simulink model "writeWord"  (Simulink 7.6)
settings: Solver=FixedStepDiscrete  StartTime=0.0  StopTime=10.0  FixedStep=0.001  RelTol=1e-3
libraries: simulink x17, dsPICdrivers x6
settings Model: Creator=ij8977  LastModifiedBy=ij8977
settings OptimizationCC: OptimizeModelRefInitCode=on  LifeSpan=1
settings RTWCC: SystemTargetFile=pic32.tlc  TemplateMakefile=pic32_gcc.tmf  PostCodeGenCommand=dsPIC_Compile()  Description=Embedded Target for Microchip dsPIC (real-time)  ProcessScript=pic32_make_rtw_hook
settings CodeAppCC: IgnoreCustomStorageClasses=off
settings STFCustomTargetCC: IncludeMdlTerminateFcn=off  CombineOutputUpdateFcns=on  SuppressErrorStatus=on  ERTCustomFileBanners=on  SupportContinuousTime=off  SupportNonInlinedSFcns=off  SystemTargetFile=pic32.tlc
settings ERTTargetCC: MultiwordLength=2048  ParMdlRefBuildCompliant=off  CompOptLevelCompliant=off  IncludeMdlTerminateFcn=off  SuppressErrorStatus=on  ERTFirstTimeCompliant=off  ModelStepFunctionPrototypeControlCompliant=off  CPPClassGenCompliant=off  InlinedParameterPlacement=NonHierarchical  ERTSrcFileBannerTemplate=dsPIC_code_template.cgt  ERTHdrFileBannerTemplate=dsPIC_code_template.cgt  ERTDataSrcFileTemplate=dsPIC_code_template.cgt  ERTDataHdrFileTemplate=dsPIC_code_template.cgt  ERTCustomFileTemplate=dsPIC_main.tlc  ConvertIfToSwitch=off
settings CustomProperty: DataType=string  Value=C:\PROGRA~1\MATLAB\R2010b\bin\win32\gmake

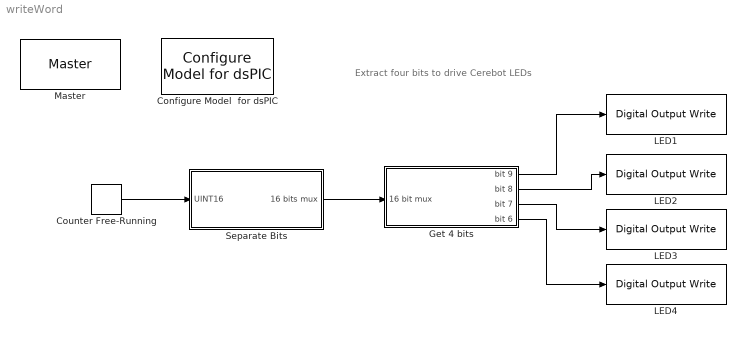
== system writeWord ==
  note: Extract four bits to drive Cerebot LEDs
  Configure Model  for dsPIC : dsPICdrivers/Simulink Configuration/Configure Model  for dsPIC
  Counter Free-Running : simulink/Sources/Counter Free-Running  SystemSampleTime=-1  NumBits=16  tsamp=-1
  Get 4 bits : Subsystem
  LED1 : dsPICdrivers/Digital I//O/Digital Output Write  Tag=dsPIC_Digital_Output  Priority=5  PORT=B  Pin=[10]  Simultaneous=off  OrderingInOutPopup=None
  LED2 : dsPICdrivers/Digital I//O/Digital Output Write  Tag=dsPIC_Digital_Output  Priority=5  PORT=B  Pin=[11]  Simultaneous=off  OrderingInOutPopup=None
  LED3 : dsPICdrivers/Digital I//O/Digital Output Write  Tag=dsPIC_Digital_Output  Priority=5  PORT=B  Pin=[12]  Simultaneous=off  OrderingInOutPopup=None
  LED4 : dsPICdrivers/Digital I//O/Digital Output Write  Tag=dsPIC_Digital_Output  Priority=5  PORT=B  Pin=[13]  Simultaneous=off  OrderingInOutPopup=None
  Master : dsPICdrivers/Master  Tag=dsPIC_MASTER  Priority=1  TimeStepType=Timer1  picType=32MX460F512L  fcy=80000000  Quartz_33f=8e6  PLLActive_33f=on  fcyDesired_33f=80e6  tmr1="[8  9999  0]"  tmr1Info="Time Step : 0.001  ;   Error : 0%  PR1=9999"  tmr2345="[0  0  0  0]"  tmr2345cfg=[-1 -1 -1 -1]  IOautoConf=on  typePort="[ 0   0   0   0   0   0   0   0   0   0   0   0   0   0   0   0   0   0   0   0   0   0   0   0   0   0  10  10  10  10   0   0   0   0   0   0   0   0   0   0   0   0   0   0   0   0   0   0   0   0   0   0   0   0   0   0   0   0   0   0   0   0   0   0   0   0   0   0   0   0   0   0   0   0   0   0   0   0   0   0   0   0   0   0   0   0   0   0   0   0   0   0   0   0   0   0   0   0   0   0   0   0   0   0   0   0   0   0   0   0   0   0 ]"  TRIS="[ 65535  50175  65535  65535  65535  65535  65535 ]"  ADPCFG=15360  MasterBusyPort=None  MasterOverloadPort=None  FOSC=Quartz (XT - HS)  ClockSwitchMonitor=Both disabled  TempProtection_33f=TEMP_ON  FPBOR=<empty>  PWRT=disable  MCLR=<empty>  ICD=ICS_NONE  JTAGEN=JTAGEN_OFF  PowerSave=off  OverrideFcy=off  NewFcy=1e6  PR2345="[65535  65535  65535  65535]"
  Separate Bits : Subsystem
  wires:
  Counter Free-Running/1 -> Separate Bits/1(UINT16)
  Get 4 bits/1(bit 9) -> LED1/1
  Get 4 bits/2(bit 8) -> LED2/1
  Get 4 bits/3(bit 7) -> LED3/1
  Get 4 bits/4(bit 6) -> LED4/1
  Separate Bits/1(16 bits mux) -> Get 4 bits/1(16 bit mux)

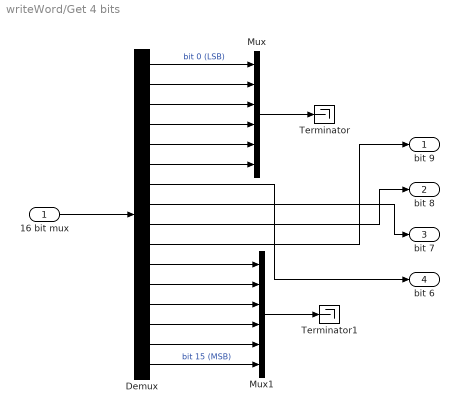
== system writeWord/Get 4 bits ==
  16 bit mux : Inport
  Demux : Demux  Outputs=16
  Mux : Mux  Inputs=6
  Mux1 : Mux  Inputs=6
  Terminator : Terminator
  Terminator1 : Terminator
  bit 9 : Outport
  bit 8 : Outport  Port=2
  bit 7 : Outport  Port=3
  bit 6 : Outport  Port=4
  wires:
  Mux/1 -> Terminator/1
  Demux/1 -> Mux/1  "bit 0 (LSB)"
  Demux/2 -> Mux/2
  Demux/3 -> Mux/3
  Demux/4 -> Mux/4
  Demux/5 -> Mux/5
  Demux/6 -> Mux/6
  Mux1/1 -> Terminator1/1
  Demux/11 -> Mux1/1
  Demux/12 -> Mux1/2
  Demux/13 -> Mux1/3
  Demux/14 -> Mux1/4
  Demux/15 -> Mux1/5
  Demux/16 -> Mux1/6  "bit 15 (MSB)"
  Demux/7 -> bit 6/1
  Demux/8 -> bit 7/1
  Demux/9 -> bit 8/1
  Demux/10 -> bit 9/1
  16 bit mux/1 -> Demux/1

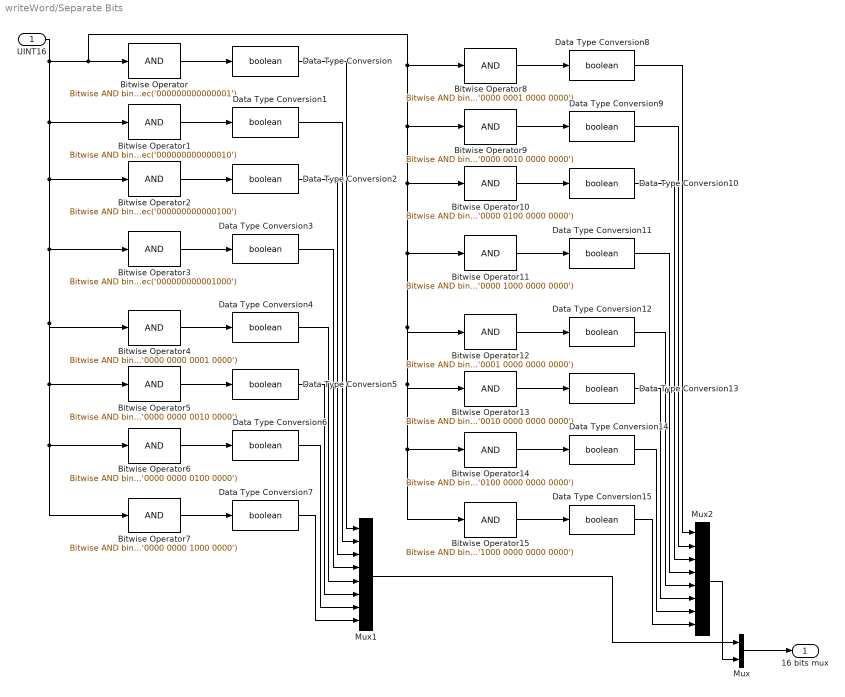
== system writeWord/Separate Bits ==
  UINT16 : Inport
  Bitwise Operator : simulink/Logic and Bit Operations/Bitwise Operator  logicop=AND  UseBitMask=on  BitMask=bin2dec('000000000000001')  BitMaskRealWorld=Stored Integer
  Bitwise Operator1 : simulink/Logic and Bit Operations/Bitwise Operator  logicop=AND  UseBitMask=on  BitMask=bin2dec('000000000000010')  BitMaskRealWorld=Stored Integer
  Bitwise Operator10 : simulink/Logic and Bit Operations/Bitwise Operator  logicop=AND  UseBitMask=on  BitMask=bin2dec('0000 0100 0000 0000')  BitMaskRealWorld=Stored Integer
  Bitwise Operator11 : simulink/Logic and Bit Operations/Bitwise Operator  logicop=AND  UseBitMask=on  BitMask=bin2dec('0000 1000 0000 0000')  BitMaskRealWorld=Stored Integer
  Bitwise Operator12 : simulink/Logic and Bit Operations/Bitwise Operator  logicop=AND  UseBitMask=on  BitMask=bin2dec('0001 0000 0000 0000')  BitMaskRealWorld=Stored Integer
  Bitwise Operator13 : simulink/Logic and Bit Operations/Bitwise Operator  logicop=AND  UseBitMask=on  BitMask=bin2dec('0010 0000 0000 0000')  BitMaskRealWorld=Stored Integer
  Bitwise Operator14 : simulink/Logic and Bit Operations/Bitwise Operator  logicop=AND  UseBitMask=on  BitMask=bin2dec('0100 0000 0000 0000')  BitMaskRealWorld=Stored Integer
  Bitwise Operator15 : simulink/Logic and Bit Operations/Bitwise Operator  logicop=AND  UseBitMask=on  BitMask=bin2dec('1000 0000 0000 0000')  BitMaskRealWorld=Stored Integer
  Bitwise Operator2 : simulink/Logic and Bit Operations/Bitwise Operator  logicop=AND  UseBitMask=on  BitMask=bin2dec('000000000000100')  BitMaskRealWorld=Stored Integer
  Bitwise Operator3 : simulink/Logic and Bit Operations/Bitwise Operator  logicop=AND  UseBitMask=on  BitMask=bin2dec('000000000001000')  BitMaskRealWorld=Stored Integer
  Bitwise Operator4 : simulink/Logic and Bit Operations/Bitwise Operator  logicop=AND  UseBitMask=on  BitMask=bin2dec('0000 0000 0001 0000')  BitMaskRealWorld=Stored Integer
  Bitwise Operator5 : simulink/Logic and Bit Operations/Bitwise Operator  logicop=AND  UseBitMask=on  BitMask=bin2dec('0000 0000 0010 0000')  BitMaskRealWorld=Stored Integer
  Bitwise Operator6 : simulink/Logic and Bit Operations/Bitwise Operator  logicop=AND  UseBitMask=on  BitMask=bin2dec('0000 0000 0100 0000')  BitMaskRealWorld=Stored Integer
  Bitwise Operator7 : simulink/Logic and Bit Operations/Bitwise Operator  logicop=AND  UseBitMask=on  BitMask=bin2dec('0000 0000 1000 0000')  BitMaskRealWorld=Stored Integer
  Bitwise Operator8 : simulink/Logic and Bit Operations/Bitwise Operator  logicop=AND  UseBitMask=on  BitMask=bin2dec('0000 0001 0000 0000')  BitMaskRealWorld=Stored Integer
  Bitwise Operator9 : simulink/Logic and Bit Operations/Bitwise Operator  logicop=AND  UseBitMask=on  BitMask=bin2dec('0000 0010 0000 0000')  BitMaskRealWorld=Stored Integer
  Data Type Conversion{,1..15} (16 alike) : DataTypeConversion  OutDataTypeStr=boolean
  Mux : Mux  Inputs=2
  Mux1 : Mux  Inputs=8
  Mux2 : Mux  Inputs=8
  16 bits mux : Outport
  wires:
  UINT16/1 -> Bitwise Operator1/1, Bitwise Operator7/1, Bitwise Operator6/1, Bitwise Operator5/1, Bitwise Operator4/1, Bitwise Operator3/1, Bitwise Operator2/1, Bitwise Operator/1, Bitwise Operator15/1, Bitwise Operator14/1, Bitwise Operator13/1, Bitwise Operator12/1, Bitwise Operator11/1, Bitwise Operator10/1, Bitwise Operator9/1, Bitwise Operator8/1
  Bitwise Operator/1 -> Data Type Conversion/1
  Data Type Conversion/1 -> Mux1/1
  Data Type Conversion1/1 -> Mux1/2
  Data Type Conversion2/1 -> Mux1/3
  Data Type Conversion3/1 -> Mux1/4
  Data Type Conversion4/1 -> Mux1/5
  Data Type Conversion5/1 -> Mux1/6
  Data Type Conversion6/1 -> Mux1/7
  Data Type Conversion7/1 -> Mux1/8
  Mux1/1 -> Mux/1
  Mux/1 -> 16 bits mux/1
  Bitwise Operator1/1 -> Data Type Conversion1/1
  Bitwise Operator2/1 -> Data Type Conversion2/1
  Bitwise Operator3/1 -> Data Type Conversion3/1
  Bitwise Operator4/1 -> Data Type Conversion4/1
  Bitwise Operator5/1 -> Data Type Conversion5/1
  Bitwise Operator6/1 -> Data Type Conversion6/1
  Bitwise Operator7/1 -> Data Type Conversion7/1
  Bitwise Operator8/1 -> Data Type Conversion8/1
  Data Type Conversion8/1 -> Mux2/1
  Data Type Conversion9/1 -> Mux2/2
  Data Type Conversion10/1 -> Mux2/3
  Data Type Conversion11/1 -> Mux2/4
  Data Type Conversion12/1 -> Mux2/5
  Data Type Conversion13/1 -> Mux2/6
  Data Type Conversion14/1 -> Mux2/7
  Data Type Conversion15/1 -> Mux2/8
  Bitwise Operator9/1 -> Data Type Conversion9/1
  Bitwise Operator10/1 -> Data Type Conversion10/1
  Bitwise Operator11/1 -> Data Type Conversion11/1
  Bitwise Operator12/1 -> Data Type Conversion12/1
  Bitwise Operator13/1 -> Data Type Conversion13/1
  Bitwise Operator14/1 -> Data Type Conversion14/1
  Bitwise Operator15/1 -> Data Type Conversion15/1
  Mux2/1 -> Mux/2
